simulink model "BSB_PI_Regler_sim"  (R2026b)
settings: Solver=VariableStepAuto  StopTime=300  FixedStep=0.001  MaxStep=0.01  MinStep=0.001
libraries: slpidlib x1
settings Model: SimulationMode=accelerator  Creator=Enrico  LastModifiedBy=Enrico

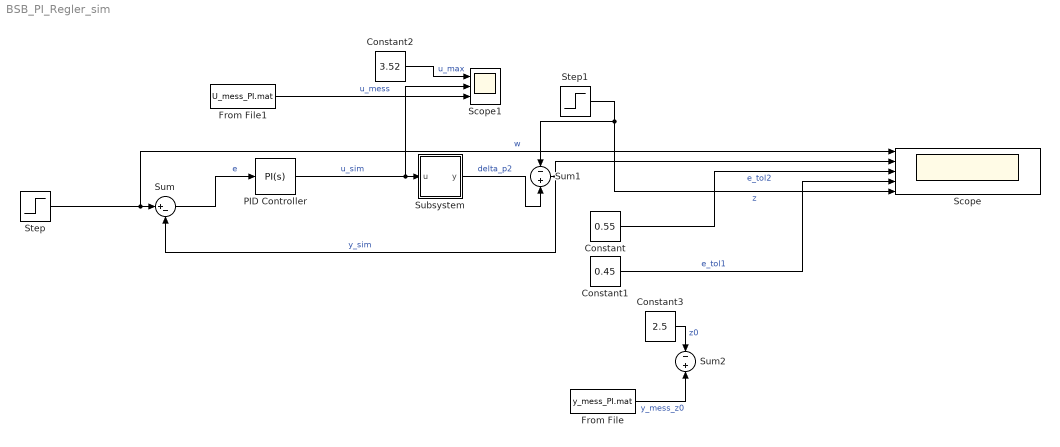
== system BSB_PI_Regler_sim ==
  Constant : Constant  Value=0.55
  Constant1 : Constant  Value=0.45
  Constant2 : Constant  Value=3.52
  Constant3 : Constant  Value=2.5
  From File : FromFile  FileName=y_mess_PI.mat  SampleTime=0
  From File1 : FromFile  FileName=U_mess_PI.mat  SampleTime=0
  PID Controller : slpidlib/PID Controller  Controller=PI  Form=Parallel  TimeDomain=Continuous-time  UseExternalTs=off  SampleTime=-1  IntegratorMethod=Forward Euler  FilterMethod=Forward Euler  ControllerParametersSource=internal  P=4.85  I=0.67  UseKiTs=off  D=0  UseExternalDerivativeSource=off  N=100  UseFilter=on  TunerSelectOption=Transfer Function Based (PID Tuner App)  InitialConditionSource=internal  InitialConditionForIntegrator=0  InitialConditionForFilter=0  DifferentiatorICPrevScaledInput=0  ExternalReset=none  TrackingMode=off  Kt=1  LimitOutput=off  SatLimitsSource=internal  UpperSaturationLimit=inf  LowerSaturationLimit=-inf  LinearizeAsGain=on  AntiWindupMode=none  Kb=1  LimitIntegrator=off  UpperIntegratorSaturationLimit=inf  LowerIntegratorSaturationLimit=-inf  POutMin=[]  POutMax=[]  IOutMin=[]  IOutMax=[]  DOutMin=[]  DOutMax=[]  NOutMin=[]  NOutMax=[]  SumOutMin=[]  SumOutMax=[]  SaturationOutMin=[]  SaturationOutMax=[]  PParamMin=[]  PParamMax=[]  IParamMin=[]  IParamMax=[]  DParamMin=[]  DParamMax=[]  NParamMin=[]  NParamMax=[]  KbParamMin=[]  KbParamMax=[]  KtParamMin=[]  KtParamMax=[]  KbOutMin=[]  KbOutMax=[]  KtOutMin=[]  KtOutMax=[]  IntegratorOutMin=[]  IntegratorOutMax=[]  FilterOutMin=[]  FilterOutMax=[]  SumI1OutMin=[]  SumI1OutMax=[]  SumI2OutMin=[]  SumI2OutMax=[]  SumI3OutMin=[]  SumI3OutMax=[]  SumI4OutMin=[]  SumI4OutMax=[]  SumDOutMin=[]  SumDOutMax=[]  DifferentiatorOutMin=[]  DifferentiatorOutMax=[]  FilterDiffOutCoefMin=[]  FilterDiffOutCoefMax=[]  ReciprocalOutMin=[]  ReciprocalOutMax=[]  SumDenOutMin=[]  SumDenOutMax=[]  SumNumOutMin=[]  SumNumOutMax=[]  DivideOutMin=[]  DivideOutMax=[]  UdiffTsProdOutMin=[]  UdiffTsProdOutMax=[]  NTsProdOutMin=[]  NTsProdOutMax=[]  UintegralTsProdOutMin=[]  UintegralTsProdOutMax=[]  UngainTsProdOutMin=[]  UngainTsProdOutMax=[]  ClampingZeroOutDataTypeStr=Inherit: Inherit via back propagation  ClampingZeroOutMin=[]  ClampingZeroOutMax=[]  FilterDenConstantOutDataTypeStr=Inherit: Inherit via back propagation  FilterDenConstantOutMin=[]  FilterDenConstantOutMax=[]  PCopyOutDataTypeStr=Inherit: Inherit via back propagation  PCopyOutMin=[]  PCopyOutMax=[]  NCopyOutDataTypeStr=Inherit: Inherit via back propagation  NCopyOutMin=[]  NCopyOutMax=[]  IntegratorContinuousStateAttributes=''  IntegratorStateMustResolveToSignalObject=off  IntegratorRTWStateStorageClass=Auto  FilterContinuousStateAttributes=''  FilterStateMustResolveToSignalObject=off  FilterRTWStateStorageClass=Auto  ParallelPVariant=InternalParameters  IdealPVariant=Disabled  IVariant=InternalParameters  DVariant=Disabled  IntegratorVariant=Continuous  SatVariant=Disabled  AWVariant=Passthrough  PCopyVariant=Disabled  TRVariant=Disabled  FdbkBlocksVariant=Forward  IdealPFdbkVariant=Disabled  SatFdbkVariant=Disabled  DerivativeFilterVariant=Disabled  NVariant=Disabled  NCopyVariant=Disabled_SignalSpec  FilterICVariant=Disabled  IntegratorICVariant=InternalICs  ExternalResetVariant=Disabled  TRSumVariant=Passthrough  SumFdbkVariant=Disabled  SumVariant=Sum_PI  TsampFilterVariant=InternalTs  TsampNgainVariant=Passthrough  TsampIntegralVariant=Disabled_SignalSpec  ExternalSaturationOutDataTypeStr=Inherit: Same as second input  DerivativeSourceVariant=Disabled  PreIntVariant=InternalPreInt
  Scope : Scope  NumInputPorts=5
      settings: ActiveDisplayYMinimum=-0.32064948841648677  ActiveDisplayYMaximum=0.54222509670759034  DataLoggingMaxPoints=100000
  Scope1 : Scope  NumInputPorts=3
      settings: ActiveDisplayYMinimum=3.4829171693173158  ActiveDisplayYMaximum=3.5234469346003587
  Step : Step  Time=100  FinalValue=0.5  SampleTime=0
  Step1 : Step  Time=200  FinalValue=0.5  SampleTime=0
  Subsystem : Subsystem  mask{Ks=0.54, Ta=1.5, Tb=10.5}
  Sum : Sum  Inputs=|+-
  Sum1 : Sum  Inputs=-+
  Sum2 : Sum  Inputs=-+
  wires:
  Constant1/1 -> Scope/4  "e_tol1"
  Constant/1 -> Scope/3  "e_tol2"
  Subsystem/1(y) -> Sum1/2  "delta_p2"
  Sum/1 -> PID Controller/1  "e"
  PID Controller/1 -> Scope1/2, Subsystem/1(u)  "u_sim"
  Step/1 -> Scope/1, Sum/1  "w"
  Step1/1 -> Scope/5, Sum1/1  "z"
  Sum1/1 -> Sum/2, Scope/2  "y_sim"
  Constant2/1 -> Scope1/1  "u_max"
  From File/1 -> Sum2/2  "y_mess_z0"
  Constant3/1 -> Sum2/1  "z0"
  From File1/1 -> Scope1/3  "u_mess"

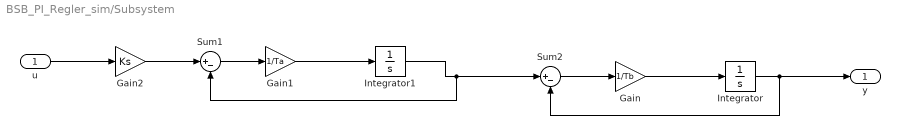
== system BSB_PI_Regler_sim/Subsystem ==
  u : Inport
  Gain : Gain  Gain=1/Tb
  Gain1 : Gain  Gain=1/Ta
  Gain2 : Gain  Gain=Ks
  Integrator : Integrator
  Integrator1 : Integrator
  Sum1 : Sum  Inputs=|+-
  Sum2 : Sum  Inputs=|+-
  y : Outport
  wires:
  Integrator/1 -> y/1, Sum2/2
  u/1 -> Gain2/1
  Gain1/1 -> Integrator1/1
  Sum1/1 -> Gain1/1
  Gain/1 -> Integrator/1
  Integrator1/1 -> Sum2/1, Sum1/2
  Sum2/1 -> Gain/1
  Gain2/1 -> Sum1/1
